simulink model "PMSM_VF_2level"  (R2023b)
settings: Solver=ode23tb  StartTime=0.0  StopTime=0.4  FixedStep=Ts  RelTol=1e-3  EnableMultiTasking=on
InitFcn:
  | Ts = 10e-6;
libraries: spsDCVoltageSourceLib x1, spsPermanentMagnetSynchronousMachineLib x1, simulink x1, spsUniversalBridgeLib x1, sps_lib x1
settings Model: Creator=Administrator  LastModifiedBy=123
settings SolverCC: AlgebraicLoopSolver=TrustRegion
settings DataIOCC: LimitDataPoints=on  SaveFormat=Array  SignalLoggingSaveFormat=ModelDataLogs  ReturnWorkspaceOutputs=off
settings OptimizationCC: ExpressionDepthLimit=2147483647  InitFltsAndDblsToZero=on  LifeSpan=inf
settings DebuggingCC: SaveWithParameterizedLinksMsg=none  UnderspecifiedInitializationDetection=Classic  MergeDetectMultiDrivingBlocksExec=none  SolverPrmCheckMsg=warning  FcnCallInpInsideContextMsg=warning  UnconnectedInputMsg=warning  UnconnectedOutputMsg=warning  UnconnectedLineMsg=warning  StateNameClashWarn=warning  SFUnexpectedBacktrackingDiag=warning  SFNoUnconditionalDefaultTransitionDiag=warning  SFExecutionAtInitializationDiag=none  ArithmeticOperatorsInVariantConditions=warning
settings HardwareCC: ProdBitPerPointer=32  ProdBitPerSizeT=32  ProdBitPerPtrDiffT=32  ProdLargestAtomicFloat=None  ProdIntDivRoundTo=Undefined  ProdEndianess=Unspecified  ProdWordSize=32  ProdHWDeviceType=32-bit Generic
settings ModelReferenceCC: EnableRefExpFcnMdlSchedulingChecks=on  PropagateSignalLabelsOutOfModel=off
settings SFSimCC: SimUseLocalCustomCode=off  SimParseCustomCode=off  CustomCodeUndefinedFunction=UseInterfaceOnly
settings RTWCC: RTWUseLocalCustomCode=off
settings CodeAppCC: StateflowObjectComments=on
settings GRTTargetCC: TargetFcnLib=ansi_tfl_tmw.mat  TargetLangStandard=C89/C90 (ANSI)  CombineOutputUpdateFcns=off  GRTInterface=on
settings ConfigComp: CovMetricSettings=dw  CovSaveCumulativeToWorkspaceVar=on  CovSaveSingleToWorkspaceVar=on  CovExternalEMLEnable=off

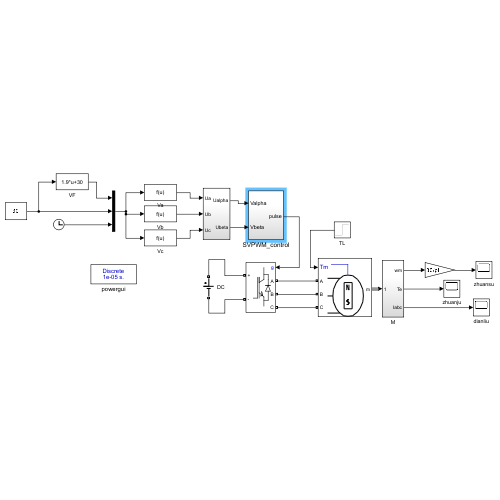
[thumbnail: Simulink's stored preview of the top-level diagram]
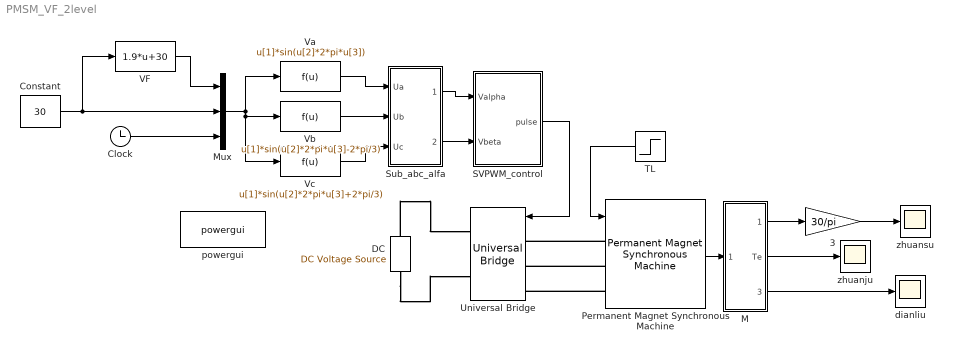
== system PMSM_VF_2level ==
  3 : Gain  Gain=30/pi
  Clock : Clock
  Constant : Constant  Value=30
  "DC " : spsDCVoltageSourceLib/DC Voltage Source  Amplitude=560  Measurements=None
  M : Subsystem
  Mux : Mux  Inputs=3
  Permanent Magnet Synchronous Machine : spsPermanentMagnetSynchronousMachineLib/Permanent Magnet Synchronous Machine  NbPhases=3  FluxDistribution=Sinusoidal  RotorType=Salient-pole  MechanicalLoad=Torque Tm  PresetModel="16:  111 Nm 560 Vdc 3000 RPM - 126 Nm"  ShowDetailedParameters=on  MeasurementBus=off  Resistance=0.05  Inductance=8.5e-3  dqInductances=[0.0006033 0.0006668]  La=0.000395  MachineConstant=Flux linkage established by magnets (V.s)  Flux=0.192  VoltageCst=139.2998  TorqueCst=1.152  Flat=120  Mechanical=[0.011 0.001889 4 0]  PolePairs=4  InitialConditions=[0,0, 0,0]  InitialConditions5ph=[0 0 0 0 0 0]  RefAngle=90 degrees behind phase A axis (modified Park)  IterativeDiscreteModel=Trapezoidal non iterative  TsBlock=-1  TsPowergui=0
  SVPWM_control : Subsystem
  Sub_abc_alfa : Subsystem
  TL : Step  Time=0.2  After=10  SampleTime=0
  Universal Bridge : spsUniversalBridgeLib/Universal Bridge  Arms=3  SnubberResistance=1e5  SnubberCapacitance=inf  Device=IGBT / Diodes  Ron=1e-3  Lon=0  ForwardVoltages="[  0  0  ]"  ForwardVoltage=0  GTOparameters=[ 10e-6 , 20e-6 ]  IGBTparameters=[ 1e-6 , 2e-6 ]  Measurements=None  Measurements_2=None  converterType=Rectifier
  VF : Fcn  Expr=1.9*u+30
  Va : Fcn  Expr=u[1]*sin(u[2]*2*pi*u[3])
  Vb : Fcn  Expr=u[1]*sin(u[2]*2*pi*u[3]-2*pi/3)
  Vc : Fcn  Expr=u[1]*sin(u[2]*2*pi*u[3]+2*pi/3)
  dianliu : Scope
  powergui : sps_lib/powergui  SimulationMode=Discrete  SampleTime=Ts  frequency=60  Iterations=50  frequencyindice=0  Pbase=100e6  ErrMax=1e-4  UnitsV=kV  UnitsW=MW  buscounter=0  FunctionMessages=off  echomessages=off  EnableUseOfTLC=off  CurrentSourceSwitches=off  DisableSnubberDevices=off  DisableRonSwitches=off  DisableVfSwitches=off  DisplayEquations=off  AutomaticDiscreteSolvers=off  SolverType=Tustin/Backward Euler (TBE)  Interpol=off  ExternalGateDelay=off  methode=off  Ts=0  x0status=blocks  SPID=off  SwTol=0  HookPort=off  NonlinearTolerance=1e-4  nMaxIteration=100  ContinueOnMaxIteration=off  RestoreLinks=warning  ResistiveCurrentMeasurement=off  Frange=[0:2:500]  Ylog=off  Xlog=on  ShowGrid=off  save=off  variable=ZData  structure=0  ZoomFFT=off  StartTime=0.0  cycles=1  DisplayStyle=1  fundamental=60  FreqAxis=off  MaxFrequency=1000  frequencyindicesteady=1  RmsSteady=1  display=off
  zhuanju : Scope
  zhuansu : Scope
  wires:
  Permanent Magnet Synchronous Machine/1 -> M/1(In1)
  M/2(Te) -> zhuanju/1
  TL/1 -> Permanent Magnet Synchronous Machine/1
  M/1(wm) -> 3/1
  Constant/1 -> Mux/2, VF/1
  M/3(Iabc) -> dianliu/1
  3/1 -> zhuansu/1
  Mux/1 -> Va/1, Vb/1, Vc/1
  VF/1 -> Mux/1
  Clock/1 -> Mux/3
  Sub_abc_alfa/1(Ualpha) -> SVPWM_control/1(Valpha)
  Sub_abc_alfa/2(Ubeta) -> SVPWM_control/2(Vbeta)
  Vb/1 -> Sub_abc_alfa/2(Ub)
  Vc/1 -> Sub_abc_alfa/3(Uc)
  Va/1 -> Sub_abc_alfa/1(Ua)
  SVPWM_control/1(pulse) -> Universal Bridge/1
  connections:
  "DC "/RConn1 -- Universal Bridge/RConn1
  "DC "/LConn1 -- Universal Bridge/RConn2
  Permanent Magnet Synchronous Machine/LConn1 -- Universal Bridge/LConn1
  Permanent Magnet Synchronous Machine/LConn2 -- Universal Bridge/LConn2
  Permanent Magnet Synchronous Machine/LConn3 -- Universal Bridge/LConn3

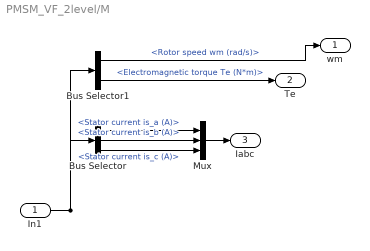
== system PMSM_VF_2level/M ==
  In1 : Inport
  Bus Selector : BusSelector  OutputSignals=Stator current is_a (A),Stator current is_b (A),Stator current is_c (A)
  Bus Selector1 : BusSelector  OutputSignals=Rotor speed wm (rad/s),Rotor angle thetam (rad),Electromagnetic torque Te (N*m)
  Mux : Mux  Inputs=3
  wm : Outport
  Te : Outport  Port=2
  Iabc : Outport  Port=3
  wires:
  Bus Selector/1 -> Mux/1  "<Stator current is_a (A)>"
  Bus Selector/2 -> Mux/2  "<Stator current is_b (A)>"
  Bus Selector/3 -> Mux/3  "<Stator current is_c (A)>"
  Bus Selector1/1 -> wm/1  "<Rotor speed wm (rad/s)>"
  In1/1 -> Bus Selector1/1, Bus Selector/1
  Bus Selector1/3 -> Te/1  "<Electromagnetic torque Te (N*m)>"
  Mux/1 -> Iabc/1

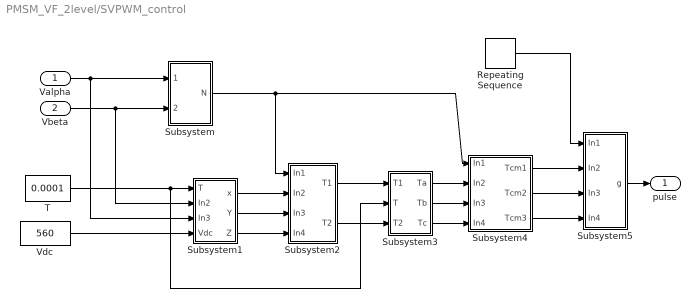
== system PMSM_VF_2level/SVPWM_control ==
  Valpha : Inport
  Vbeta : Inport  Port=2
  Repeating Sequence : simulink/Sources/Repeating Sequence  rep_seq_t=[0 0.00005 0.0001]  rep_seq_y=[0 0.00005 0]
  Subsystem : Subsystem
  Subsystem1 : Subsystem
  Subsystem2 : Subsystem
  Subsystem3 : Subsystem
  Subsystem4 : Subsystem
  Subsystem5 : Subsystem
  T : Constant  Value=0.0001
  Vdc : Constant  Value=560
  pulse : Outport
  wires:
  Subsystem5/1(g) -> pulse/1
  Repeating Sequence/1 -> Subsystem5/1(In1)
  Subsystem4/3(Tcm3) -> Subsystem5/4(In4)
  Subsystem4/2(Tcm2) -> Subsystem5/3(In3)
  Subsystem4/1(Tcm1) -> Subsystem5/2(In2)
  Subsystem3/3(Tc) -> Subsystem4/4(In4)
  Subsystem3/2(Tb) -> Subsystem4/3(In3)
  Subsystem3/1(Ta) -> Subsystem4/2(In2)
  Subsystem2/2(T2) -> Subsystem3/3(T2)
  Subsystem2/1(T1) -> Subsystem3/1(T1)
  Subsystem1/3(Z) -> Subsystem2/4(In4)
  Subsystem1/2(Y) -> Subsystem2/3(In3)
  Subsystem1/1(x) -> Subsystem2/2(In2)
  Subsystem/1(N) -> Subsystem4/1(In1), Subsystem2/1(In1)
  Vdc/1 -> Subsystem1/4(Vdc)
  T/1 -> Subsystem3/2(T), Subsystem1/1(T)
  Vbeta/1 -> Subsystem1/2(In2), Subsystem/2(Vbeta)
  Valpha/1 -> Subsystem1/3(In3), Subsystem/1(Valpha)

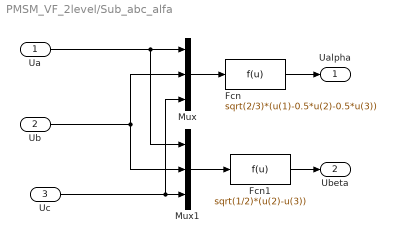
== system PMSM_VF_2level/Sub_abc_alfa ==
  Ua : Inport
  Ub : Inport  Port=2
  Uc : Inport  Port=3
  Fcn : Fcn  Expr=sqrt(2/3)*(u(1)-0.5*u(2)-0.5*u(3))
  Fcn1 : Fcn  Expr=sqrt(1/2)*(u(2)-u(3))
  Mux : Mux  Inputs=3
  Mux1 : Mux  Inputs=3
  Ualpha : Outport
  Ubeta : Outport  Port=2
  wires:
  Mux/1 -> Fcn/1
  Mux1/1 -> Fcn1/1
  Fcn/1 -> Ualpha/1
  Fcn1/1 -> Ubeta/1
  Ua/1 -> Mux/1, Mux1/1
  Uc/1 -> Mux/3, Mux1/3
  Ub/1 -> Mux/2, Mux1/2

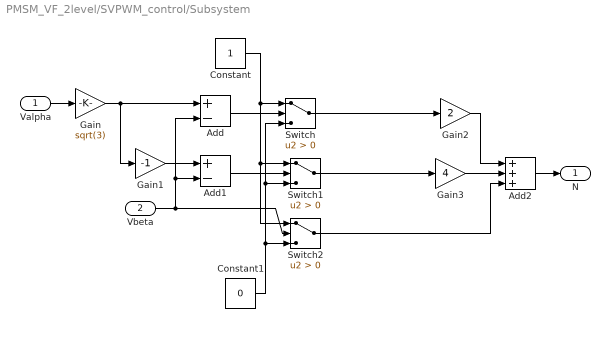
== system PMSM_VF_2level/SVPWM_control/Subsystem ==
  Valpha : Inport
  Vbeta : Inport  Port=2
  Add : Sum  Inputs=+-
  Add1 : Sum  Inputs=+-
  Add2 : Sum  Inputs=+++
  Constant : Constant
  Constant1 : Constant  Value=0
  Gain : Gain  Gain=sqrt(3)
  Gain1 : Gain  Gain=-1
  Gain2 : Gain  Gain=2
  Gain3 : Gain  Gain=4
  Switch : Switch  Criteria=u2 > Threshold  SaturateOnIntegerOverflow=off  InputSameDT=off
  Switch1 : Switch  Criteria=u2 > Threshold  SaturateOnIntegerOverflow=off  InputSameDT=off
  Switch2 : Switch  Criteria=u2 > Threshold  SaturateOnIntegerOverflow=off  InputSameDT=off
  N : Outport
  wires:
  Add2/1 -> N/1
  Valpha/1 -> Gain/1
  Gain3/1 -> Add2/2
  Gain2/1 -> Add2/1
  Add1/1 -> Switch1/2
  Gain1/1 -> Add1/1
  Switch1/1 -> Gain3/1
  Switch2/1 -> Add2/3
  Switch/1 -> Gain2/1
  Add/1 -> Switch/2
  Gain/1 -> Gain1/1, Add/1
  Constant1/1 -> Switch/3, Switch1/3, Switch2/3
  Constant/1 -> Switch1/1, Switch2/1, Switch/1
  Vbeta/1 -> Add1/2, Add/2, Switch2/2

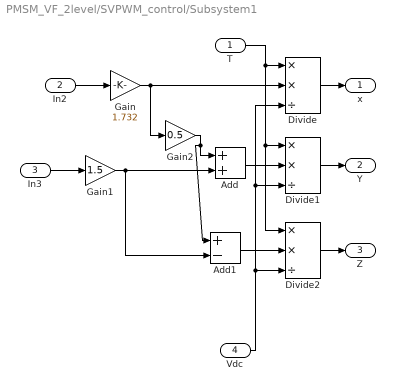
== system PMSM_VF_2level/SVPWM_control/Subsystem1 ==
  T : Inport
  In2 : Inport  Port=2
  In3 : Inport  Port=3
  Vdc : Inport  Port=4
  Add : Sum
  Add1 : Sum  Inputs=+-
  Divide : Product  Inputs=**/
  Divide1 : Product  Inputs=**/
  Divide2 : Product  Inputs=**/
  Gain : Gain  Gain=1.732
  Gain1 : Gain  Gain=1.5
  Gain2 : Gain  Gain=0.5
  x : Outport
  Y : Outport  Port=2
  Z : Outport  Port=3
  wires:
  Divide2/1 -> Z/1
  Divide1/1 -> Y/1
  Divide/1 -> x/1
  In3/1 -> Gain1/1
  In2/1 -> Gain/1
  Add1/1 -> Divide2/2
  Add/1 -> Divide1/2
  Gain1/1 -> Add1/2, Add/2
  Gain2/1 -> Add1/1, Add/1
  Gain/1 -> Gain2/1, Divide/2
  Vdc/1 -> Divide/3, Divide1/3, Divide2/3
  T/1 -> Divide2/1, Divide1/1, Divide/1

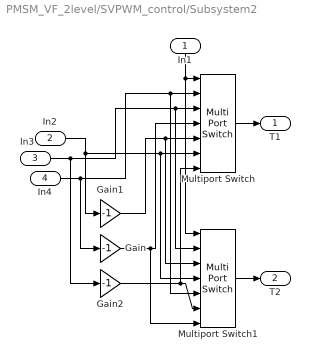
== system PMSM_VF_2level/SVPWM_control/Subsystem2 ==
  In1 : Inport
  In2 : Inport  Port=2
  In3 : Inport  Port=3
  In4 : Inport  Port=4
  Gain : Gain  Gain=-1
  Gain1 : Gain  Gain=-1
  Gain2 : Gain  Gain=-1
  Multiport Switch : MultiPortSwitch  Inputs=6  SaturateOnIntegerOverflow=off  InputSameDT=off
  Multiport Switch1 : MultiPortSwitch  Inputs=6  SaturateOnIntegerOverflow=off  InputSameDT=off
  T1 : Outport
  T2 : Outport  Port=2
  wires:
  Multiport Switch1/1 -> T2/1
  Multiport Switch/1 -> T1/1
  Gain2/1 -> Multiport Switch/7, Multiport Switch1/6
  Gain1/1 -> Multiport Switch1/3, Multiport Switch/5
  In2/1 -> Gain1/1, Multiport Switch/6, Multiport Switch1/4
  Gain/1 -> Multiport Switch1/7, Multiport Switch/4
  In3/1 -> Gain2/1, Multiport Switch1/2, Multiport Switch/3
  In4/1 -> Gain/1, Multiport Switch/2, Multiport Switch1/5
  In1/1 -> Multiport Switch/1, Multiport Switch1/1

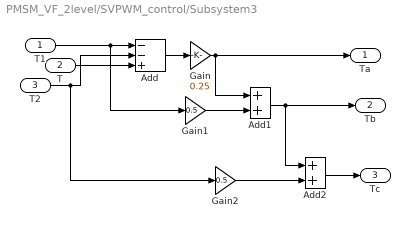
== system PMSM_VF_2level/SVPWM_control/Subsystem3 ==
  T1 : Inport
  T : Inport  Port=2
  T2 : Inport  Port=3
  Add : Sum  Inputs=--+
  Add1 : Sum
  Add2 : Sum
  Gain : Gain  Gain=0.25
  Gain1 : Gain  Gain=0.5
  Gain2 : Gain  Gain=0.5
  Ta : Outport
  Tb : Outport  Port=2
  Tc : Outport  Port=3
  wires:
  T/1 -> Add/3
  Add2/1 -> Tc/1
  Gain2/1 -> Add2/2
  Add1/1 -> Add2/1, Tb/1
  Gain1/1 -> Add1/2
  Gain/1 -> Add1/1, Ta/1
  Add/1 -> Gain/1
  T2/1 -> Add/2, Gain2/1
  T1/1 -> Add/1, Gain1/1

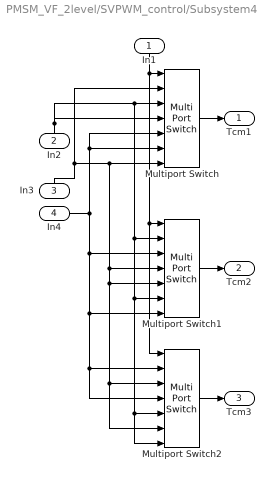
== system PMSM_VF_2level/SVPWM_control/Subsystem4 ==
  In1 : Inport
  In2 : Inport  Port=2
  In3 : Inport  Port=3
  In4 : Inport  Port=4
  Multiport Switch : MultiPortSwitch  Inputs=6  SaturateOnIntegerOverflow=off  InputSameDT=off
  Multiport Switch1 : MultiPortSwitch  Inputs=6  SaturateOnIntegerOverflow=off  InputSameDT=off
  Multiport Switch2 : MultiPortSwitch  Inputs=6  SaturateOnIntegerOverflow=off  InputSameDT=off
  Tcm1 : Outport
  Tcm2 : Outport  Port=2
  Tcm3 : Outport  Port=3
  wires:
  Multiport Switch2/1 -> Tcm3/1
  Multiport Switch1/1 -> Tcm2/1
  Multiport Switch/1 -> Tcm1/1
  In1/1 -> Multiport Switch2/1, Multiport Switch1/1, Multiport Switch/1
  In4/1 -> Multiport Switch1/3, Multiport Switch1/7, Multiport Switch2/2, Multiport Switch2/4, Multiport Switch/5, Multiport Switch/6
  In2/1 -> Multiport Switch/4, Multiport Switch/3, Multiport Switch1/2, Multiport Switch1/6, Multiport Switch2/5, Multiport Switch2/7
  In3/1 -> Multiport Switch/2, Multiport Switch/7, Multiport Switch1/4, Multiport Switch1/5, Multiport Switch2/3, Multiport Switch2/6

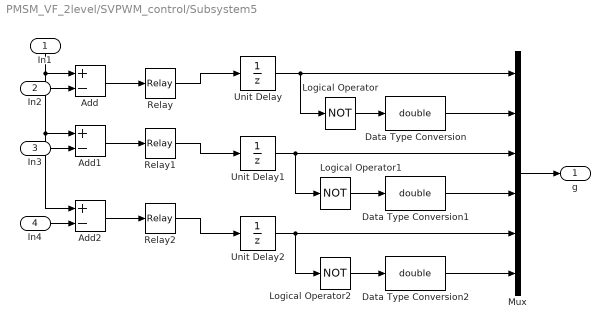
== system PMSM_VF_2level/SVPWM_control/Subsystem5 ==
  In1 : Inport
  In2 : Inport  Port=2
  In3 : Inport  Port=3
  In4 : Inport  Port=4
  Add : Sum  Inputs=+-
  Add1 : Sum  Inputs=+-
  Add2 : Sum  Inputs=+-
  Data Type Conversion : DataTypeConversion  OutDataTypeStr=double  SaturateOnIntegerOverflow=off  RndMeth=Floor
  Data Type Conversion1 : DataTypeConversion  OutDataTypeStr=double  SaturateOnIntegerOverflow=off  RndMeth=Floor
  Data Type Conversion2 : DataTypeConversion  OutDataTypeStr=double  SaturateOnIntegerOverflow=off  RndMeth=Floor
  Logical Operator : Logic  Operator=NOT  AllPortsSameDT=off  OutDataTypeStr=boolean
  Logical Operator1 : Logic  Operator=NOT  AllPortsSameDT=off  OutDataTypeStr=boolean
  Logical Operator2 : Logic  Operator=NOT  AllPortsSameDT=off  OutDataTypeStr=boolean
  Mux : Mux  Inputs=6
  Relay : Relay  OffSwitchValue=-eps
  Relay1 : Relay  OffSwitchValue=-eps
  Relay2 : Relay  OffSwitchValue=-eps
  Unit Delay : UnitDelay  SampleTime=-1
  Unit Delay1 : UnitDelay  SampleTime=-1
  Unit Delay2 : UnitDelay  SampleTime=-1
  g : Outport
  wires:
  In4/1 -> Add2/2
  In3/1 -> Add1/2
  In2/1 -> Add/2
  Relay2/1 -> Unit Delay2/1
  Relay1/1 -> Unit Delay1/1
  Relay/1 -> Unit Delay/1
  Unit Delay2/1 -> Mux/5, Logical Operator2/1
  Unit Delay1/1 -> Mux/3, Logical Operator1/1
  Unit Delay/1 -> Logical Operator/1, Mux/1
  Mux/1 -> g/1
  Data Type Conversion/1 -> Mux/2
  Data Type Conversion1/1 -> Mux/4
  Data Type Conversion2/1 -> Mux/6
  Logical Operator2/1 -> Data Type Conversion2/1
  Logical Operator1/1 -> Data Type Conversion1/1
  Logical Operator/1 -> Data Type Conversion/1
  Add1/1 -> Relay1/1
  Add2/1 -> Relay2/1
  Add/1 -> Relay/1
  In1/1 -> Add/1, Add2/1, Add1/1
